simulink library "strapnavlib"  (Simulink 5.0)
undefined symbols (not defined in the file or in its folder): skew
libraries: simulink3 x1, simulink x1
settings Model: Creator=mcar  LastModifiedBy=mcarroll  ExtModeAutoUpdateStatusClock=off

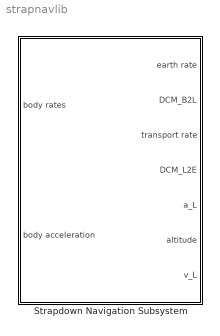
== system strapnavlib ==
  Strapdown Navigation Subsystem : Subsystem

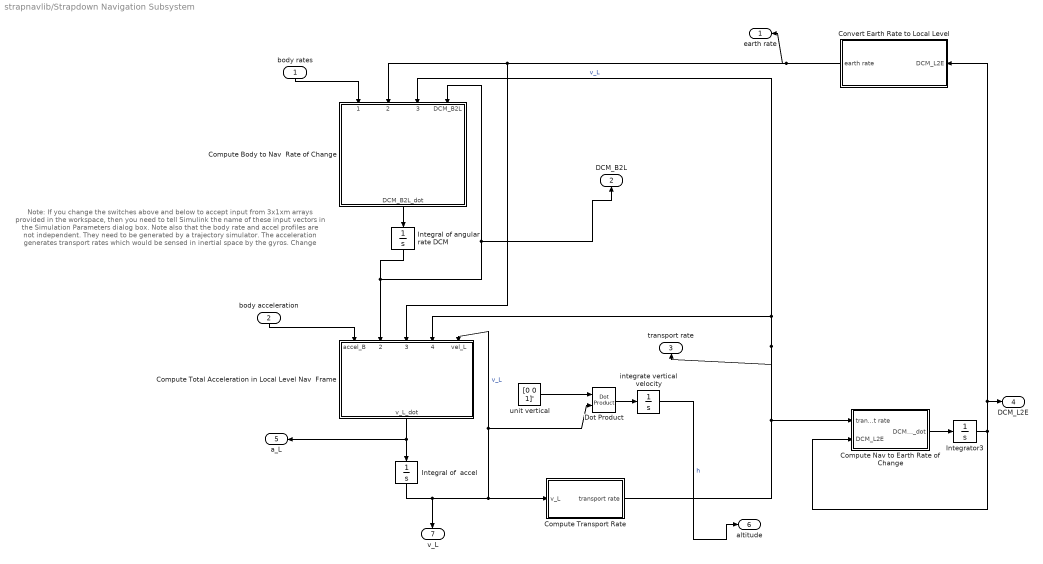
== system strapnavlib/Strapdown Navigation Subsystem ==
  note: Note: If you change
      | the switches above and below
      | to accept input from 3x1xm
      | arrays provided in the workspace, then
      | you need to tell Simulink the name of these
      | input vectors in the Simulation Parameters
      | dialog box.
      | Note also that the body rate and accel
      | profiles are not independent.  They need
      | to be generated by a trajectory simulator.
      | The acceleration generates transport rates
      | which would be sensed in inertial space
      | by the gyros.
      | Change
  body rates : Inport  Orientation=down
  body acceleration : Inport  Orientation=down  Port=2
  Compute Body to Nav  Rate of Change : Subsystem  Orientation=down
  Compute Nav to Earth Rate of Change : Subsystem
  Compute Total Acceleration in Local Level Nav  Frame : Subsystem  Orientation=down
  Compute Transport Rate : Subsystem
  Convert Earth Rate to Local Level : Subsystem  Orientation=left
  Dot Product : simulink/Math Operations/Dot Product
  Integral of angular rate DCM : Integrator  Orientation=down  InitialCondition=eye(3)
  Integral of  accel : Integrator  Orientation=down  InitialCondition=[0 0 0]'
  Integrator3 : Integrator  InitialCondition=eye(3)
  integrate vertical velocity : Integrator
  unit vertical : Constant  Value=[0 0 1]'  VectorParams1D=off
  earth rate : Outport  Orientation=left
  DCM_B2L : Outport  Orientation=up  Port=2
  transport rate : Outport  Orientation=up  Port=3
  DCM_L2E : Outport  Port=4
  a_L : Outport  Orientation=left  Port=5
  altitude : Outport  Port=6
  v_L : Outport  Orientation=down  Port=7
  wires:
  Integral of angular rate DCM/1 -> Compute Total Acceleration in Local Level Nav  Frame/2(DCM_B2L), Compute Body to Nav  Rate of Change/4(DCM_B2L), DCM_B2L/1
  Compute Body to Nav  Rate of Change/1(DCM_B2L_dot) -> Integral of angular rate DCM/1
  Compute Total Acceleration in Local Level Nav  Frame/1(v_L_dot) -> Integral of  accel/1, a_L/1
  Integral of  accel/1 -> v_L/1, Compute Transport Rate/1(v_L), Dot Product/2, Compute Total Acceleration in Local Level Nav  Frame/5(vel_L)  "v_L"
  Compute Transport Rate/1(transport rate) -> Compute Nav to Earth Rate of Change/1(transport rate), Compute Body to Nav  Rate of Change/3(transport rate), Compute Total Acceleration in Local Level Nav  Frame/4(transport rate), transport rate/1  "v_L"
  unit vertical/1 -> Dot Product/1
  Dot Product/1 -> integrate vertical velocity/1
  Compute Nav to Earth Rate of Change/1(DCM_L2E_dot) -> Integrator3/1
  Integrator3/1 -> Convert Earth Rate to Local Level/1(DCM_L2E), DCM_L2E/1, Compute Nav to Earth Rate of Change/2(DCM_L2E)
  Convert Earth Rate to Local Level/1(earth rate) -> Compute Body to Nav  Rate of Change/2(earth rate), Compute Total Acceleration in Local Level Nav  Frame/3(earth rate), earth rate/1
  integrate vertical velocity/1 -> altitude/1  "h"
  body rates/1 -> Compute Body to Nav  Rate of Change/1(body rates)
  body acceleration/1 -> Compute Total Acceleration in Local Level Nav  Frame/1(accel_B)

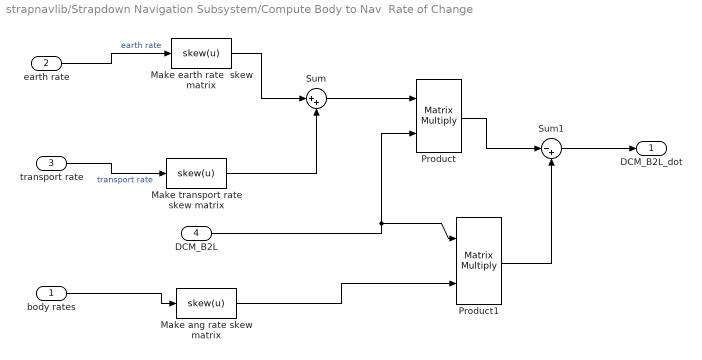
== system strapnavlib/Strapdown Navigation Subsystem/Compute Body to Nav  Rate of Change ==
  body rates : Inport
  earth rate : Inport  Port=2
  transport rate : Inport  Port=3
  DCM_B2L : Inport  Port=4
  Make ang rate skew matrix : MATLABFcn  MATLABFcn=skew(u)  Output1D=off
  Make earth rate  skew matrix : MATLABFcn  MATLABFcn=skew(u)  Output1D=off
  Make transport rate skew matrix : MATLABFcn  MATLABFcn=skew(u)  Output1D=off
  Product : Product  Multiplication=Matrix(*)  SaturateOnIntegerOverflow=on  InputSameDT=on
  Product1 : Product  Multiplication=Matrix(*)  SaturateOnIntegerOverflow=on  InputSameDT=on
  Sum : Sum  Inputs=|++  SaturateOnIntegerOverflow=on  InputSameDT=on
  Sum1 : Sum  Inputs=|-+  SaturateOnIntegerOverflow=on  InputSameDT=on
  DCM_B2L_dot : Outport
  wires:
  body rates/1 -> Make ang rate skew matrix/1
  earth rate/1 -> Make earth rate  skew matrix/1  "earth rate"
  transport rate/1 -> Make transport rate skew matrix/1  "transport rate"
  Make transport rate skew matrix/1 -> Sum/2
  Make earth rate  skew matrix/1 -> Sum/1
  DCM_B2L/1 -> Product/2, Product1/1
  Sum/1 -> Product/1
  Make ang rate skew matrix/1 -> Product1/2
  Product/1 -> Sum1/1
  Product1/1 -> Sum1/2
  Sum1/1 -> DCM_B2L_dot/1

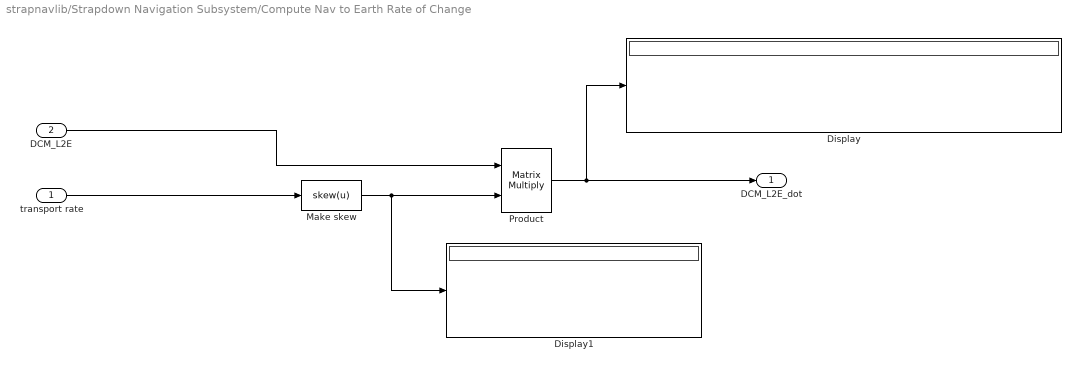
== system strapnavlib/Strapdown Navigation Subsystem/Compute Nav to Earth Rate of Change ==
  transport rate : Inport
  DCM_L2E : Inport  Port=2
  Display : Display
  Display1 : Display
  Make skew : MATLABFcn  MATLABFcn=skew(u)  Output1D=off
  Product : Product  Multiplication=Matrix(*)  SaturateOnIntegerOverflow=on  InputSameDT=on
  DCM_L2E_dot : Outport
  wires:
  Product/1 -> DCM_L2E_dot/1, Display/1
  Make skew/1 -> Product/2, Display1/1
  transport rate/1 -> Make skew/1
  DCM_L2E/1 -> Product/1

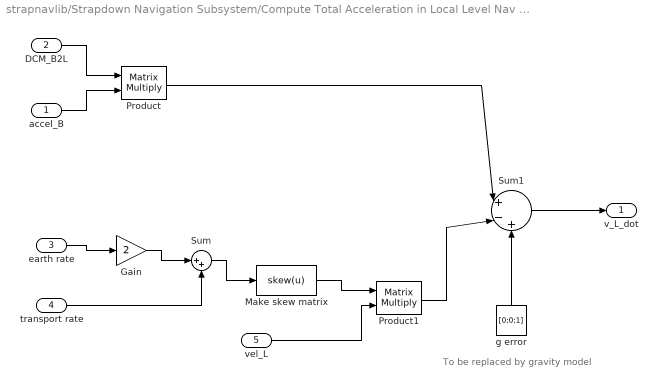
== system strapnavlib/Strapdown Navigation Subsystem/Compute Total Acceleration in Local Level Nav  Frame ==
  note: To be replaced by
      | gravity model
  accel_B : Inport
  DCM_B2L : Inport  Port=2
  earth rate : Inport  Port=3
  transport rate : Inport  Port=4
  vel_L : Inport  Port=5
  Gain : Gain  Gain=2  SaturateOnIntegerOverflow=on
  Make skew matrix : MATLABFcn  MATLABFcn=skew(u)  Output1D=off
  Product : Product  Multiplication=Matrix(*)  SaturateOnIntegerOverflow=on  InputSameDT=on
  Product1 : Product  Multiplication=Matrix(*)  SaturateOnIntegerOverflow=on  InputSameDT=on
  Sum : Sum  Inputs=|++  SaturateOnIntegerOverflow=on  InputSameDT=on
  Sum1 : Sum  Inputs=|+-+  SaturateOnIntegerOverflow=on  InputSameDT=on
  g error : Constant  Orientation=up  Value=[0;0;1]  VectorParams1D=off
  v_L_dot : Outport
  wires:
  DCM_B2L/1 -> Product/1
  accel_B/1 -> Product/2
  earth rate/1 -> Gain/1
  Gain/1 -> Sum/1
  transport rate/1 -> Sum/2
  Sum/1 -> Make skew matrix/1
  Make skew matrix/1 -> Product1/1
  vel_L/1 -> Product1/2
  Product1/1 -> Sum1/2
  g error/1 -> Sum1/3
  Product/1 -> Sum1/1
  Sum1/1 -> v_L_dot/1

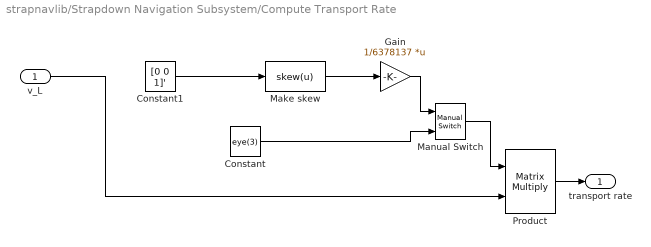
== system strapnavlib/Strapdown Navigation Subsystem/Compute Transport Rate ==
  v_L : Inport
  Constant : Constant  Value=eye(3)  VectorParams1D=off
  Constant1 : Constant  Value=[0 0 1]'  VectorParams1D=off
  Gain : Gain  Gain=1/6378137  Multiplication=Matrix(K*u)  SaturateOnIntegerOverflow=on
  Make skew : MATLABFcn  MATLABFcn=skew(u)  Output1D=off
  Manual Switch : simulink3/Nonlinear/Manual Switch  sw=1  action=0
  Product : Product  Multiplication=Matrix(*)  SaturateOnIntegerOverflow=on  InputSameDT=on
  transport rate : Outport
  wires:
  v_L/1 -> Product/2
  Constant1/1 -> Make skew/1
  Product/1 -> transport rate/1
  Constant/1 -> Manual Switch/2
  Gain/1 -> Manual Switch/1
  Make skew/1 -> Gain/1
  Manual Switch/1 -> Product/1

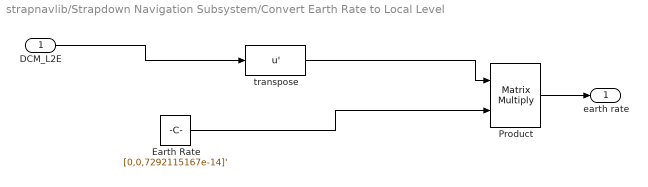
== system strapnavlib/Strapdown Navigation Subsystem/Convert Earth Rate to Local Level ==
  DCM_L2E : Inport
  Earth Rate : Constant  Value=[0,0,7292115167e-14]'  VectorParams1D=off
  Product : Product  Multiplication=Matrix(*)  SaturateOnIntegerOverflow=on  InputSameDT=on
  transpose : MATLABFcn  MATLABFcn=u'  Output1D=off
  earth rate : Outport
  wires:
  transpose/1 -> Product/1
  Product/1 -> earth rate/1
  DCM_L2E/1 -> transpose/1
  Earth Rate/1 -> Product/2
